simulink model "Model_MPC"  (R2024b)
settings: Solver=FixedStepAuto  StartTime=0.0  StopTime=10  RelTol=1e-3
undefined symbols (not defined in the file): Aa, Ba, Ca, Dm, Eyflat, Fq, Gq, k_3165_plant, k_3166_plant, L, N, qp_iter, Qref, REF_p, REF_q, tau_3165_plant, tau_3166_plant, Ts, umax, Vc_3165, Vc_3166, w, w_eps, X, x0, Y, Z
libraries: sm_lib x13, nesl_utility x5
settings Model: Creator=Giuliano Livi  LastModifiedBy=Giuliano Livi

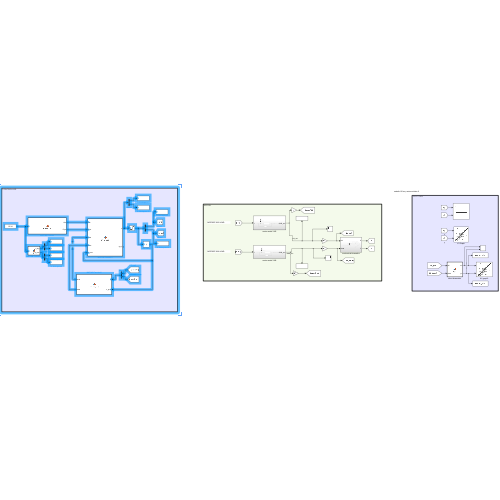
[thumbnail: Simulink's stored preview of the top-level diagram]
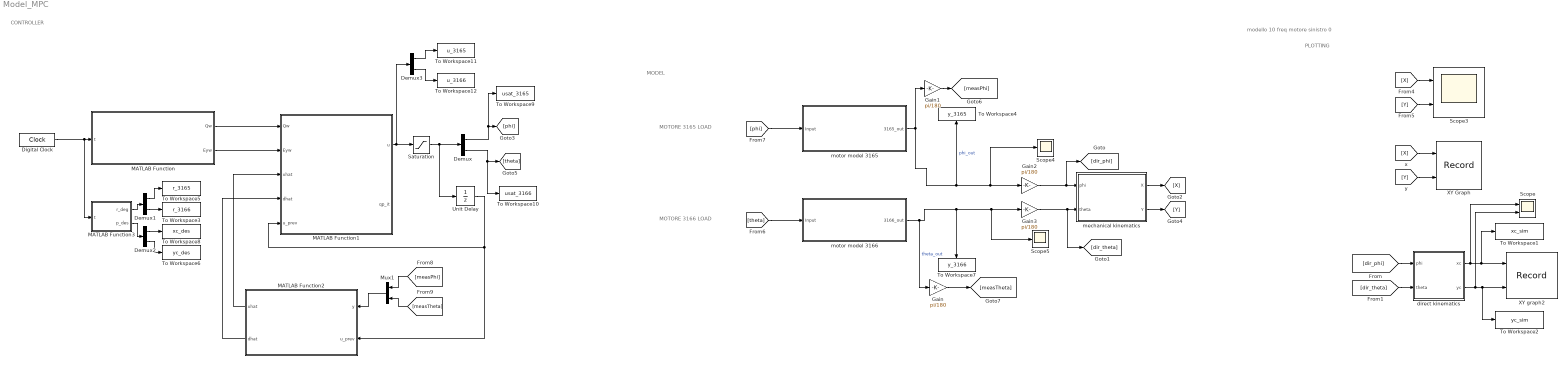
== system Model_MPC ==
  note: CONTROLLER
  note: PLOTTING
  note: MODEL
  note: MOTORE 3165 LOAD
  note: modello 10 freq motore sinistro 0
  note: MOTORE 3166 LOAD
  Demux{,1..3} (4 alike) : Demux  Outputs=2
  Digital Clock : DigitalClock  SampleTime=Ts
  Gain{,1..3} (4 alike) : Gain  Gain=pi/180
  MATLAB Function : MATLAB Function  TreatAsAtomicUnit=on
  MATLAB Function1 : MATLAB Function  TreatAsAtomicUnit=on
  MATLAB Function2 : MATLAB Function  TreatAsAtomicUnit=on
  MATLAB Function3 : MATLAB Function  TreatAsAtomicUnit=on
  Mux1 : Mux  Inputs=2
  Saturation : Saturate  UpperLimit=6  LowerLimit=-6
  Scope : Scope  NumInputPorts=2
  Scope3 : Scope  NumInputPorts=2
  Scope4 : Scope
  Scope5 : Scope
  To Workspace1 : ToWorkspace  VariableName=xc_sim  SaveFormat=Timeseries  SampleTime=0.002
  To Workspace10 : ToWorkspace  VariableName=usat_3166  SaveFormat=Timeseries  SampleTime=0.002
  To Workspace11 : ToWorkspace  VariableName=u_3165  SaveFormat=Timeseries  SampleTime=0.002
  To Workspace12 : ToWorkspace  VariableName=u_3166  SaveFormat=Timeseries  SampleTime=0.002
  To Workspace2 : ToWorkspace  VariableName=yc_sim  SaveFormat=Timeseries  SampleTime=0.002
  To Workspace3 : ToWorkspace  VariableName=r_3166  SaveFormat=Timeseries  SampleTime=0.002
  To Workspace4 : ToWorkspace  VariableName=y_3165  SaveFormat=Timeseries  SampleTime=0.002
  To Workspace5 : ToWorkspace  VariableName=r_3165  SaveFormat=Timeseries  SampleTime=0.002
  To Workspace6 : ToWorkspace  VariableName=yc_des  SaveFormat=Timeseries  SampleTime=0.002
  To Workspace7 : ToWorkspace  VariableName=y_3166  SaveFormat=Timeseries  SampleTime=0.002
  To Workspace8 : ToWorkspace  VariableName=xc_des  SaveFormat=Timeseries  SampleTime=0.002
  To Workspace9 : ToWorkspace  VariableName=usat_3165  SaveFormat=Timeseries  SampleTime=0.002
  Unit Delay : UnitDelay  SampleTime=Ts  HasFrameUpgradeWarning=on
  XY Graph : Record  FileSettingsInternal="{\"entries\":[{\"content\":{\"excelSettings\":{\"content\":{},\"type\":\"Streamout.ExcelSettings\"}},\"type\":\"Streamout.FileSettingStorage\",\"uuid\":\"\"}],\"packageUris\":[\"http:\\/\\/schema.mathworks.com\\/mf0\\/streamout_blocks\\/R2020a\"],\"version\":\"1.0\"}"  Layout=[1 1]  SignalsInternal="{\"entries\":[{\"content\":{\"signals\":[{\"content\":{\"blockPath\":[],\"dimensions\":[1],\"domain\":\"\",\"lineColor\":\"#a2142f\",\"plots\":[ 1 ],\"port\":1,\"sid\":[\"\"],\"signalID\":1,\"signalName\":\"x\"},\"type\":\"RecordBlkView.Signal\",\"uuid\":\"\"},{\"content\":{\"blockPath\":[],\"dimensions\":[1],\"domain\":\"\",\"lineColor\":\"#139fff\",\"plots\":[ 1 ],\"port\":2,\"sid\":[\"\"],\"signalID\":2,\"signalName\":\"y\"},\"type\":\"RecordBlkView.Signal\",\"uuid\":\"\"}]},\"type\":\"RecordBlkView.InputSignals\",\"uuid\":\"\"}],\"packageUris\":[\"http:\\/\\/schema.mathworks.com\\/mf0\\/streamout_blocks\\/R2020a\"],\"version\":\"1.0\"}"  VisualizationBindings="{\"xyplotplugin\":{\"info\":[{\"series\":[{\"bindingParametersList\":[{\"parameter\":\"X-Axis\",\"signalID\":1,\"signalName\":\"x\"},{\"parameter\":\"Y-Axis\",\"signalID\":2,\"signalName\":\"y\"}],\"seriesID\":0}],\"subplotID\":1}]}}"  CompatibilityTag=XY
  XY graph2 : Record  FileSettingsInternal="{\"entries\":[{\"content\":{\"excelSettings\":{\"content\":{},\"type\":\"Streamout.ExcelSettings\"}},\"type\":\"Streamout.FileSettingStorage\",\"uuid\":\"\"}],\"packageUris\":[\"http:\\/\\/schema.mathworks.com\\/mf0\\/streamout_blocks\\/R2020a\"],\"version\":\"1.0\"}"  Layout=[1 1]  SignalsInternal="{\"entries\":[{\"content\":{\"signals\":[{\"content\":{\"blockPath\":[],\"dimensions\":[1],\"domain\":\"\",\"lineColor\":\"#a2142f\",\"lineWidth\":2,\"plots\":[ 1 ],\"port\":1,\"sid\":[\"\"],\"signalID\":1,\"signalName\":\"direct kinematics:1\"},\"type\":\"RecordBlkView.Signal\",\"uuid\":\"\"},{\"content\":{\"blockPath\":[],\"dimensions\":[1],\"domain\":\"\",\"lineColor\":\"#139fff\",\"lineWidth\":2,\"plots\":[ 1 ],\"port\":2,\"sid\":[\"\"],\"signalID\":2,\"signalName\":\"direct kinematics:2\"},\"type\":\"RecordBlkView.Signal\",\"uuid\":\"\"}]},\"type\":\"RecordBlkView.InputSignals\",\"uuid\":\"\"}],\"packageUris\":[\"http:\\/\\/schema.mathworks.com\\/mf0\\/streamout_blocks\\/R2020a\"],\"version\":\"1.0\"}"  VisualizationBindings="{\"xyplotplugin\":{\"info\":[{\"series\":[{\"bindingParametersList\":[{\"parameter\":\"X-Axis\",\"signalID\":1,\"signalName\":\"direct kinematics:1\"},{\"parameter\":\"Y-Axis\",\"signalID\":2,\"signalName\":\"direct kinematics:2\"}],\"seriesID\":0},{\"bindingParametersList\":[{\"parameter\":\"X-Axis\",\"signalID\":1,\"signalName\":\"direct kinematics:1\"},{\"parameter\":\"Y-Axis\",\"signalID\":2,\"signalName\":\"direct kinematics:2\"}],\"seriesID\":1}],\"subplotID\":1}]}}"  CompatibilityTag=XY
  direct kinematics : MATLAB Function  TreatAsAtomicUnit=on  SystemSampleTime=0.002
  mechanical kinematics : Subsystem
  motor model 3165 : Subsystem
  motor model 3166 : Subsystem
  wires:
  Gain2/1 -> mechanical kinematics/1(phi), [dir_phi]
  [X] -> Scope3/1
  [X] -> XY Graph/1
  direct kinematics/2(yc) -> Scope/2, To Workspace2/1, XY graph2/2
  [dir_theta] -> direct kinematics/2(theta)
  motor model 3166/1(3166_out) -> Gain/1, To Workspace7/1, Gain3/1, Scope5/1  "theta_out"
  direct kinematics/1(xc) -> Scope/1, To Workspace1/1, XY graph2/1
  mechanical kinematics/2(Y) -> [Y]
  Gain3/1 -> [dir_theta], mechanical kinematics/2(theta)
  motor model 3165/1(3165_out) -> Gain2/1, Scope4/1, To Workspace4/1, Gain1/1  "phi_out"
  [Y] -> Scope3/2
  mechanical kinematics/1(X) -> [X]
  [phi] -> motor model 3165/1(Input)
  [Y] -> XY Graph/2
  [dir_phi] -> direct kinematics/1(phi)
  [theta] -> motor model 3166/1(Input)
  Digital Clock/1 -> MATLAB Function3/1(t), MATLAB Function/1(t)
  MATLAB Function/2(Eyw) -> MATLAB Function1/2(Eyw)
  MATLAB Function2/1(xhat) -> MATLAB Function1/3(xhat)
  MATLAB Function2/2(dhat) -> MATLAB Function1/4(dhat)
  MATLAB Function1/1(u) -> Saturation/1, Demux3/1
  Saturation/1 -> Unit Delay/1, Demux/1
  Demux/1 -> To Workspace9/1, [phi]
  Demux/2 -> To Workspace10/1, [theta]
  MATLAB Function/1(Qw) -> MATLAB Function1/1(Qw)
  Mux1/1 -> MATLAB Function2/1(y)
  [measPhi] -> Mux1/1
  [measTheta] -> Mux1/2
  Unit Delay/1 -> MATLAB Function2/2(u_prev), MATLAB Function1/5(u_prev)
  Gain/1 -> [measTheta]
  Gain1/1 -> [measPhi]
  MATLAB Function3/1(r_deg) -> Demux1/1
  Demux1/1 -> To Workspace5/1
  Demux1/2 -> To Workspace3/1
  MATLAB Function3/2(p_des) -> Demux2/1
  Demux2/1 -> To Workspace8/1
  Demux2/2 -> To Workspace6/1
  Demux3/1 -> To Workspace11/1
  Demux3/2 -> To Workspace12/1

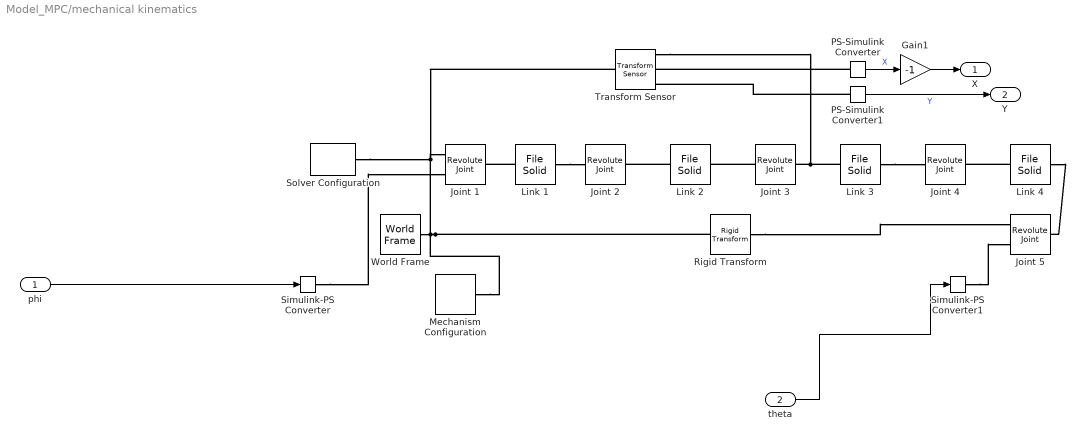
== system Model_MPC/mechanical kinematics ==
  phi : Inport
  theta : Inport  Port=2
  Gain1 : Gain  Gain=-1
  Joint 1 : sm_lib/Joints/Revolute Joint  JointMode=Normal  CompositeWrenchDir=FollowerOnBase  CompositeWrenchFrame=BaseFrame  SenseConstraintForce=off  SenseConstraintTorque=off  SenseTotalForce=off  SenseTotalTorque=off  PositionTargetSpecify=off  PositionTargetPriority=High  PositionTargetValue=0  PositionTargetValueUnits=deg  VelocityTargetSpecify=off  VelocityTargetPriority=High  VelocityTargetValue=0  VelocityTargetValueUnits=deg/s  EquilibriumPosition=0  EquilibriumPositionUnits=deg  SpringStiffness=0  SpringStiffnessUnits=N*m/deg  DampingCoefficient=0  DampingCoefficientUnits=N*m/(deg/s)  LowerLimitSpecify=off  LowerLimitBound=-90  LowerLimitBoundUnits=deg  LowerLimitStiffness=1e4  LowerLimitStiffnessUnits=N*m/deg  LowerLimitDamping=10  LowerLimitDampingUnits=N*m/(deg/s)  LowerLimitTransitionRegionWidth=0.1  LowerLimitTransitionRegionWidthUnits=deg  UpperLimitSpecify=off  UpperLimitBound=90  UpperLimitBoundUnits=deg  UpperLimitStiffness=1e4  UpperLimitStiffnessUnits=N*m/deg  UpperLimitDamping=10  UpperLimitDampingUnits=N*m/(deg/s)  UpperLimitTransitionRegionWidth=0.1  UpperLimitTransitionRegionWidthUnits=deg  TorqueActuationMode=ComputedTorque  MotionActuationMode=InputMotion  SensePosition=off  SenseVelocity=off  SenseAcceleration=off  SenseTorqueForce=off  SenseLowerLimitTorqueForce=off  SenseUpperLimitTorqueForce=off
  Joint 2 : sm_lib/Joints/Revolute Joint  JointMode=Normal  CompositeWrenchDir=FollowerOnBase  CompositeWrenchFrame=BaseFrame  SenseConstraintForce=off  SenseConstraintTorque=off  SenseTotalForce=off  SenseTotalTorque=off  PositionTargetSpecify=off  PositionTargetPriority=High  PositionTargetValue=90  PositionTargetValueUnits=deg  VelocityTargetSpecify=off  VelocityTargetPriority=High  VelocityTargetValue=0  VelocityTargetValueUnits=deg/s  EquilibriumPosition=0  EquilibriumPositionUnits=deg  SpringStiffness=0  SpringStiffnessUnits=N*m/deg  DampingCoefficient=0  DampingCoefficientUnits=N*m/(deg/s)  LowerLimitSpecify=off  LowerLimitBound=-90  LowerLimitBoundUnits=deg  LowerLimitStiffness=1e4  LowerLimitStiffnessUnits=N*m/deg  LowerLimitDamping=10  LowerLimitDampingUnits=N*m/(deg/s)  LowerLimitTransitionRegionWidth=0.1  LowerLimitTransitionRegionWidthUnits=deg  UpperLimitSpecify=off  UpperLimitBound=90  UpperLimitBoundUnits=deg  UpperLimitStiffness=1e4  UpperLimitStiffnessUnits=N*m/deg  UpperLimitDamping=10  UpperLimitDampingUnits=N*m/(deg/s)  UpperLimitTransitionRegionWidth=0.1  UpperLimitTransitionRegionWidthUnits=deg  TorqueActuationMode=NoTorque  MotionActuationMode=ComputedMotion  SensePosition=off  SenseVelocity=off  SenseAcceleration=off  SenseTorqueForce=off  SenseLowerLimitTorqueForce=off  SenseUpperLimitTorqueForce=off
  Joint 3 : sm_lib/Joints/Revolute Joint  JointMode=Normal  CompositeWrenchDir=FollowerOnBase  CompositeWrenchFrame=BaseFrame  SenseConstraintForce=off  SenseConstraintTorque=off  SenseTotalForce=off  SenseTotalTorque=off  PositionTargetSpecify=off  PositionTargetPriority=High  PositionTargetValue=0  PositionTargetValueUnits=deg  VelocityTargetSpecify=off  VelocityTargetPriority=High  VelocityTargetValue=0  VelocityTargetValueUnits=deg/s  EquilibriumPosition=0  EquilibriumPositionUnits=deg  SpringStiffness=0  SpringStiffnessUnits=N*m/deg  DampingCoefficient=0  DampingCoefficientUnits=N*m/(deg/s)  LowerLimitSpecify=off  LowerLimitBound=-90  LowerLimitBoundUnits=deg  LowerLimitStiffness=1e4  LowerLimitStiffnessUnits=N*m/deg  LowerLimitDamping=10  LowerLimitDampingUnits=N*m/(deg/s)  LowerLimitTransitionRegionWidth=0.1  LowerLimitTransitionRegionWidthUnits=deg  UpperLimitSpecify=off  UpperLimitBound=90  UpperLimitBoundUnits=deg  UpperLimitStiffness=1e4  UpperLimitStiffnessUnits=N*m/deg  UpperLimitDamping=10  UpperLimitDampingUnits=N*m/(deg/s)  UpperLimitTransitionRegionWidth=0.1  UpperLimitTransitionRegionWidthUnits=deg  TorqueActuationMode=NoTorque  MotionActuationMode=ComputedMotion  SensePosition=off  SenseVelocity=off  SenseAcceleration=off  SenseTorqueForce=off  SenseLowerLimitTorqueForce=off  SenseUpperLimitTorqueForce=off
  Joint 4 : sm_lib/Joints/Revolute Joint  JointMode=Normal  CompositeWrenchDir=FollowerOnBase  CompositeWrenchFrame=BaseFrame  SenseConstraintForce=off  SenseConstraintTorque=off  SenseTotalForce=off  SenseTotalTorque=off  PositionTargetSpecify=off  PositionTargetPriority=High  PositionTargetValue=0  PositionTargetValueUnits=deg  VelocityTargetSpecify=off  VelocityTargetPriority=High  VelocityTargetValue=0  VelocityTargetValueUnits=deg/s  EquilibriumPosition=0  EquilibriumPositionUnits=deg  SpringStiffness=0  SpringStiffnessUnits=N*m/deg  DampingCoefficient=0  DampingCoefficientUnits=N*m/(deg/s)  LowerLimitSpecify=off  LowerLimitBound=-90  LowerLimitBoundUnits=deg  LowerLimitStiffness=1e4  LowerLimitStiffnessUnits=N*m/deg  LowerLimitDamping=10  LowerLimitDampingUnits=N*m/(deg/s)  LowerLimitTransitionRegionWidth=0.1  LowerLimitTransitionRegionWidthUnits=deg  UpperLimitSpecify=off  UpperLimitBound=90  UpperLimitBoundUnits=deg  UpperLimitStiffness=1e4  UpperLimitStiffnessUnits=N*m/deg  UpperLimitDamping=10  UpperLimitDampingUnits=N*m/(deg/s)  UpperLimitTransitionRegionWidth=0.1  UpperLimitTransitionRegionWidthUnits=deg  TorqueActuationMode=NoTorque  MotionActuationMode=ComputedMotion  SensePosition=off  SenseVelocity=off  SenseAcceleration=off  SenseTorqueForce=off  SenseLowerLimitTorqueForce=off  SenseUpperLimitTorqueForce=off
  Joint 5 : sm_lib/Joints/Revolute Joint  JointMode=Normal  CompositeWrenchDir=FollowerOnBase  CompositeWrenchFrame=BaseFrame  SenseConstraintForce=off  SenseConstraintTorque=off  SenseTotalForce=off  SenseTotalTorque=off  PositionTargetSpecify=off  PositionTargetPriority=High  PositionTargetValue=0  PositionTargetValueUnits=deg  VelocityTargetSpecify=off  VelocityTargetPriority=High  VelocityTargetValue=0  VelocityTargetValueUnits=deg/s  EquilibriumPosition=0  EquilibriumPositionUnits=deg  SpringStiffness=0  SpringStiffnessUnits=N*m/deg  DampingCoefficient=0  DampingCoefficientUnits=N*m/(deg/s)  LowerLimitSpecify=off  LowerLimitBound=-90  LowerLimitBoundUnits=deg  LowerLimitStiffness=1e4  LowerLimitStiffnessUnits=N*m/deg  LowerLimitDamping=10  LowerLimitDampingUnits=N*m/(deg/s)  LowerLimitTransitionRegionWidth=0.1  LowerLimitTransitionRegionWidthUnits=deg  UpperLimitSpecify=off  UpperLimitBound=90  UpperLimitBoundUnits=deg  UpperLimitStiffness=1e4  UpperLimitStiffnessUnits=N*m/deg  UpperLimitDamping=10  UpperLimitDampingUnits=N*m/(deg/s)  UpperLimitTransitionRegionWidth=0.1  UpperLimitTransitionRegionWidthUnits=deg  TorqueActuationMode=ComputedTorque  MotionActuationMode=InputMotion  SensePosition=off  SenseVelocity=off  SenseAcceleration=off  SenseTorqueForce=off  SenseLowerLimitTorqueForce=off  SenseUpperLimitTorqueForce=off
  Link 1 : sm_lib/Body Elements/File Solid  ExtGeomFileName=link.step  UnitType=FromFile  ExtGeomFileUnits=m  StepReaderType=HEX  ExportConvexHullGeometry=off  InertiaType=CalculateFromGeometry  BasedOnType=Mass  Density=1000  DensityUnits=kg/m^3  Mass=0.065  MassUnits=kg  CenterOfMass=[0 0 0]  CenterOfMassUnits=m  MomentsOfInertia=[1 1 1]  MomentsOfInertiaUnits=kg*m^2  ProductsOfInertia=[0 0 0]  ProductsOfInertiaUnits=kg*m^2  GraphicType=FromGeometry  MarkerShape=Sphere  MarkerSize=10  GraphicVisPropType=SimpleVisualProperties  GraphicDiffuseColor=[0.5 0.5 0.5]  GraphicOpacity=1  GraphicSpecularColor=[0.5 0.5 0.5 1.0]  GraphicAmbientColor=[0.15 0.15 0.15 1.0]  GraphicEmissiveColor=[0.0 0.0 0.0 1.0]  GraphicShininess=75  DoExposeReferenceFrame=off  SerializedFrames=<Frames><Frame><Id>Frame1</Id><Value><Name>F1</Name><Origin><Source>GeometricFeature</Source><FeatureName>cylindrical surface 1</FeatureName></Origin><PrimaryAxis><DefinedDirection>+Z</DefinedDirection><Source>ReferenceFrame</Source><SourceDirection>+Z</SourceDirection><FeatureName></FeatureName></PrimaryAxis><SecondaryAxis><DefinedDirection>+Y</DefinedDirection><Source>ReferenceFrame</Source><SourceDirection>+X</SourceDirection><FeatureName></FeatureName></SecondaryAxis></Value></Frame><Frame><Id>Frame2</Id><Value><Name>F2</Name><Origin><Source>GeometricFeature</Source><FeatureName>cylindrical surface 2</FeatureName></Origin><PrimaryAxis><DefinedDirection>+Z</DefinedDirection><Source>ReferenceFrame</Source><SourceDirection>+Z</SourceDirection><FeatureName></FeatureName></PrimaryAxis><SecondaryAxis><DefinedDirection>+X</DefinedDirection><Source>ReferenceFrame</Source><SourceDirection>+X</SourceDirection><FeatureName></FeatureName></SecondaryAxis></Value></Frame></Frames>
  Link 2 : sm_lib/Body Elements/File Solid  ExtGeomFileName=link.step  UnitType=FromFile  ExtGeomFileUnits=m  StepReaderType=HEX  ExportConvexHullGeometry=off  InertiaType=CalculateFromGeometry  BasedOnType=Mass  Density=1000  DensityUnits=kg/m^3  Mass=0.065  MassUnits=kg  CenterOfMass=[0 0 0]  CenterOfMassUnits=m  MomentsOfInertia=[1 1 1]  MomentsOfInertiaUnits=kg*m^2  ProductsOfInertia=[0 0 0]  ProductsOfInertiaUnits=kg*m^2  GraphicType=FromGeometry  MarkerShape=Sphere  MarkerSize=10  GraphicVisPropType=SimpleVisualProperties  GraphicDiffuseColor=[0.5 0.5 0.5]  GraphicOpacity=1  GraphicSpecularColor=[0.5 0.5 0.5 1.0]  GraphicAmbientColor=[0.15 0.15 0.15 1.0]  GraphicEmissiveColor=[0.0 0.0 0.0 1.0]  GraphicShininess=75  DoExposeReferenceFrame=off  SerializedFrames=<Frames><Frame><Id>Frame1</Id><Value><Name>F1</Name><Origin><Source>GeometricFeature</Source><FeatureName>cylindrical surface 1</FeatureName></Origin><PrimaryAxis><DefinedDirection>+Z</DefinedDirection><Source>ReferenceFrame</Source><SourceDirection>+Z</SourceDirection><FeatureName></FeatureName></PrimaryAxis><SecondaryAxis><DefinedDirection>+X</DefinedDirection><Source>ReferenceFrame</Source><SourceDirection>+X</SourceDirection><FeatureName></FeatureName></SecondaryAxis></Value></Frame><Frame><Id>Frame2</Id><Value><Name>F2</Name><Origin><Source>GeometricFeature</Source><FeatureName>cylindrical surface 2</FeatureName></Origin><PrimaryAxis><DefinedDirection>+Z</DefinedDirection><Source>ReferenceFrame</Source><SourceDirection>+Z</SourceDirection><FeatureName></FeatureName></PrimaryAxis><SecondaryAxis><DefinedDirection>+X</DefinedDirection><Source>ReferenceFrame</Source><SourceDirection>+X</SourceDirection><FeatureName></FeatureName></SecondaryAxis></Value></Frame></Frames>
  Link 3 : sm_lib/Body Elements/File Solid  ExtGeomFileName=link.step  UnitType=FromFile  ExtGeomFileUnits=m  StepReaderType=HEX  ExportConvexHullGeometry=off  InertiaType=CalculateFromGeometry  BasedOnType=Mass  Density=1000  DensityUnits=kg/m^3  Mass=0.065  MassUnits=kg  CenterOfMass=[0 0 0]  CenterOfMassUnits=m  MomentsOfInertia=[1 1 1]  MomentsOfInertiaUnits=kg*m^2  ProductsOfInertia=[0 0 0]  ProductsOfInertiaUnits=kg*m^2  GraphicType=FromGeometry  MarkerShape=Sphere  MarkerSize=10  GraphicVisPropType=SimpleVisualProperties  GraphicDiffuseColor=[0.5 0.5 0.5]  GraphicOpacity=1  GraphicSpecularColor=[0.5 0.5 0.5 1.0]  GraphicAmbientColor=[0.15 0.15 0.15 1.0]  GraphicEmissiveColor=[0.0 0.0 0.0 1.0]  GraphicShininess=75  DoExposeReferenceFrame=off  SerializedFrames=<Frames><Frame><Id>Frame1</Id><Value><Name>F1</Name><Origin><Source>GeometricFeature</Source><FeatureName>cylindrical surface 1</FeatureName></Origin><PrimaryAxis><DefinedDirection>+Z</DefinedDirection><Source>ReferenceFrame</Source><SourceDirection>+Z</SourceDirection><FeatureName></FeatureName></PrimaryAxis><SecondaryAxis><DefinedDirection>+X</DefinedDirection><Source>ReferenceFrame</Source><SourceDirection>+X</SourceDirection><FeatureName></FeatureName></SecondaryAxis></Value></Frame><Frame><Id>Frame2</Id><Value><Name>F2</Name><Origin><Source>GeometricFeature</Source><FeatureName>cylindrical surface 2</FeatureName></Origin><PrimaryAxis><DefinedDirection>+Z</DefinedDirection><Source>ReferenceFrame</Source><SourceDirection>+Z</SourceDirection><FeatureName></FeatureName></PrimaryAxis><SecondaryAxis><DefinedDirection>+X</DefinedDirection><Source>ReferenceFrame</Source><SourceDirection>+X</SourceDirection><FeatureName></FeatureName></SecondaryAxis></Value></Frame></Frames>
  Link 4 : sm_lib/Body Elements/File Solid  ExtGeomFileName=link.step  UnitType=FromFile  ExtGeomFileUnits=m  StepReaderType=HEX  ExportConvexHullGeometry=off  InertiaType=CalculateFromGeometry  BasedOnType=Mass  Density=1000  DensityUnits=kg/m^3  Mass=0.065  MassUnits=kg  CenterOfMass=[0 0 0]  CenterOfMassUnits=m  MomentsOfInertia=[1 1 1]  MomentsOfInertiaUnits=kg*m^2  ProductsOfInertia=[0 0 0]  ProductsOfInertiaUnits=kg*m^2  GraphicType=FromGeometry  MarkerShape=Sphere  MarkerSize=10  GraphicVisPropType=SimpleVisualProperties  GraphicDiffuseColor=[0.5 0.5 0.5]  GraphicOpacity=1  GraphicSpecularColor=[0.5 0.5 0.5 1.0]  GraphicAmbientColor=[0.15 0.15 0.15 1.0]  GraphicEmissiveColor=[0.0 0.0 0.0 1.0]  GraphicShininess=75  DoExposeReferenceFrame=off  SerializedFrames=<Frames><Frame><Id>Frame1</Id><Value><Name>F1</Name><Origin><Source>GeometricFeature</Source><FeatureName>cylindrical surface 1</FeatureName></Origin><PrimaryAxis><DefinedDirection>+Z</DefinedDirection><Source>ReferenceFrame</Source><SourceDirection>+Z</SourceDirection><FeatureName></FeatureName></PrimaryAxis><SecondaryAxis><DefinedDirection>+X</DefinedDirection><Source>ReferenceFrame</Source><SourceDirection>+X</SourceDirection><FeatureName></FeatureName></SecondaryAxis></Value></Frame><Frame><Id>Frame2</Id><Value><Name>F2</Name><Origin><Source>GeometricFeature</Source><FeatureName>cylindrical surface 2</FeatureName></Origin><PrimaryAxis><DefinedDirection>+Z</DefinedDirection><Source>ReferenceFrame</Source><SourceDirection>+Z</SourceDirection><FeatureName></FeatureName></PrimaryAxis><SecondaryAxis><DefinedDirection>+X</DefinedDirection><Source>ReferenceFrame</Source><SourceDirection>+X</SourceDirection><FeatureName></FeatureName></SecondaryAxis></Value></Frame></Frames>
  Mechanism Configuration : sm_lib/Utilities/Mechanism Configuration  UniformGravity=Constant  GravityVector=[0 0 -9.80665]  GravityVectorUnits=m/s^2  LinearizationDelta=0.001  JointModeTransitionNonlinearIterations=2
  PS-Simulink Converter : nesl_utility/PS-Simulink Converter  PhysicalDomain=network_engine_domain  SubClassName=ps_output  LeftPortType=input  RightPortType=output  PseudoPeriodic=off  Frequencies=[]  VectorFormat=inherit  Unit=inherit  AffineConversion=off
  PS-Simulink Converter1 : nesl_utility/PS-Simulink Converter  PhysicalDomain=network_engine_domain  SubClassName=ps_output  LeftPortType=input  RightPortType=output  PseudoPeriodic=off  Frequencies=[]  VectorFormat=inherit  Unit=inherit  AffineConversion=off
  Rigid Transform : sm_lib/Frames and Transforms/Rigid Transform  RotationMethod=None  FollAlignAxisA=+X  BaseAlignAxisA=+Y  FollAlignAxisB=+Y  BaseAlignAxisB=+Z  RotationStandardAxis=+Z  RotationAngle=0  RotationAngleUnits=deg  RotationArbitraryAxis=[0 0 1]  RotationSequenceAxes=FollowerAxes  RotationSequence=XYX  RotationSequenceAngles=[0 0 0]  RotationSequenceAnglesUnits=deg  RotationMatrix=[1 0 0;0 1 0;0 0 1]  Quaternion=[1 0 0 0]  TranslationMethod=Cartesian  TranslationCartesianOffset=[0 0.254 0]  TranslationCartesianOffsetUnits=m  TranslationStandardAxis=+Z  TranslationStandardOffset=0  TranslationStandardOffsetUnits=m  TranslationROffset=0  TranslationROffsetUnits=m  TranslationThetaOffset=0  TranslationThetaOffsetUnits=deg  TranslationZOffset=0  TranslationZOffsetUnits=m
  Simulink-PS Converter : nesl_utility/Simulink-PS Converter  PhysicalDomain=network_engine_domain  SubClassName=ps_input  LeftPortType=input  RightPortType=output  PseudoPeriodic=off  Frequencies=[]  NoiseDistribution=none  NoiseParameters=[]  Unit=rad  AffineConversion=off  FilteringAndDerivatives=filter  SimscapeFilterOrder=2  InputFilterTimeConstant=0.001  UdotUserProvided=0
  Simulink-PS Converter1 : nesl_utility/Simulink-PS Converter  PhysicalDomain=network_engine_domain  SubClassName=ps_input  LeftPortType=input  RightPortType=output  PseudoPeriodic=off  Frequencies=[]  NoiseDistribution=none  NoiseParameters=[]  Unit=rad  AffineConversion=off  FilteringAndDerivatives=filter  SimscapeFilterOrder=2  InputFilterTimeConstant=0.001  UdotUserProvided=0
  Solver Configuration : nesl_utility/Solver Configuration  PhysicalDomain=network_engine_domain  SubClassName=solver  LeftPortType=input  RightPortType=generic  Tones=[]  Harmonics=[]  SimulateNoise=off  Profile=off  UseLocalSampling=off  EnableSwitchedLinearOptims=on  FrequencyDomain=off  UseCCode=off  RelTol=0.001  AbsTol=0.001  MinStep=1e-09  ToWorkspace=off  RevertToSquareIcSolve=off  NumHomotopyIterations=100  PhasorMode=off  PhasorModeNumHarmonics=1  ConsistencySolver=NEWTON_XTOL_AFTER_FTOL  IndexReductionMethod=DerivativeReplacement  DoDC=on  ResidualTolerance=1e-09  ConsistencyTolSource=GLOBAL  ConsistencyAbsTol=0.001  ConsistencyRelTol=0.001  ConsistencyTolFactor=0.001  UseLocalSolver=off  LocalSolverChoice=NE_BACKWARD_EULER_ADVANCER  ResolveIndetEquations=on  FunctionEvalNumThread=1  LocalSolverSampleTime=0.002  DoFixedCost=off  MaxNonlinIter=3  MaxModeIter=2  ComputeImpulses=off  ImpulseIterations=2  LinearAlgebra=auto  LinearAlgebraNumThread=0  EquationFormulation=NE_TIME_EF  DelaysMemoryBudget=1024  AutomaticFiltering=on  FilteringTimeConstant=0.001  PartitionStorageMethod=AS_NEEDED  PartitionMemoryBudget=1024  PartitionMethod=ROBUST  MultibodyUseLocalSolver=off  MultibodyLocalSolverChoice=ODE2  MultibodyLocalSolverSampleTime=0.002
  Transform Sensor : sm_lib/Frames and Transforms/Transform Sensor  MeasurementFrame=World  RotationSequence=XYX  SenseAngle=off  SenseAxis=off  SenseQ=off  SenseR=off  SenseRotationSequence=off  SenseOmegaX=off  SenseOmegaY=off  SenseOmegaZ=off  SenseOmega=off  SenseQDot=off  SenseRDot=off  SenseRotationSequenceDot=off  SenseAlphaX=off  SenseAlphaY=off  SenseAlphaZ=off  SenseAlpha=off  SenseQDDot=off  SenseRDDot=off  SenseX=on  SenseY=on  SenseZ=off  SenseXYZ=off  SenseRad=off  SenseAzim=off  SenseDist=off  SenseInc=off  SenseXDot=off  SenseYDot=off  SenseZDot=off  SenseXYZDot=off  SenseRadDot=off  SenseAzimDot=off  SenseDistDot=off  SenseIncDot=off  SenseXDDot=off  SenseYDDot=off  SenseZDDot=off  SenseXYZDDot=off  SenseRadDDot=off  SenseAzimDDot=off  SenseDistDDot=off  SenseIncDDot=off
  World Frame : sm_lib/Frames and Transforms/World Frame
  X : Outport
  Y : Outport  Port=2
  wires:
  theta/1 -> Simulink-PS Converter1/1
  phi/1 -> Simulink-PS Converter/1
  PS-Simulink Converter1/1 -> Y/1  "Y"
  PS-Simulink Converter/1 -> Gain1/1  "X"
  Gain1/1 -> X/1
  connections:
  World Frame/RConn1 -- Rigid Transform/LConn1 -- Transform Sensor/LConn1 -- Joint 1/LConn1 -- Solver Configuration/RConn1 -- Mechanism Configuration/RConn1
  Joint 3/LConn1 -- Link 2/RConn1
  Link 3/LConn1 -- Transform Sensor/RConn1 -- Joint 3/RConn1
  Simulink-PS Converter1/RConn1 -- Joint 5/LConn2
  Rigid Transform/RConn1 -- Joint 5/LConn1
  Link 3/RConn1 -- Joint 4/LConn1
  Link 1/RConn1 -- Joint 2/LConn1
  Link 4/LConn1 -- Joint 4/RConn1
  Link 4/RConn1 -- Joint 5/RConn1
  Link 2/LConn1 -- Joint 2/RConn1
  Link 1/LConn1 -- Joint 1/RConn1
  Simulink-PS Converter/RConn1 -- Joint 1/LConn2
  PS-Simulink Converter/LConn1 -- Transform Sensor/RConn2
  PS-Simulink Converter1/LConn1 -- Transform Sensor/RConn3

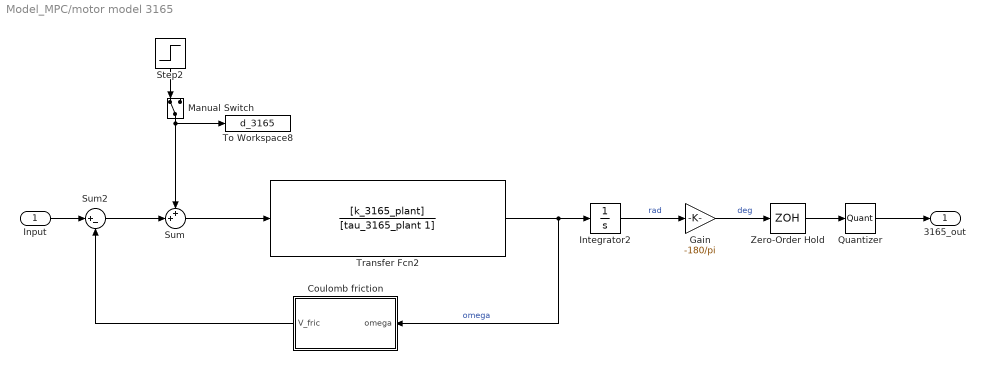
== system Model_MPC/motor model 3165 ==
  Input : Inport
  Coulomb friction : MATLAB Function  TreatAsAtomicUnit=on
  Gain : Gain  Gain=-180/pi
  Integrator2 : Integrator
  Manual Switch : ManualSwitch
  Quantizer : Quantizer  QuantizationInterval=360/4096
  Step2 : Step  Time=5  After=0.5  SampleTime=0
  Sum : Sum  Inputs=++|
  Sum2 : Sum  Inputs=|+-
  To Workspace8 : ToWorkspace  VariableName=d_3165  SaveFormat=Timeseries  SampleTime=-1
  Transfer Fcn2 : TransferFcn  Numerator=[k_3165_plant]  Denominator=[tau_3165_plant 1]
  Zero-Order Hold : ZeroOrderHold  SampleTime=0.002
  3165_out : Outport
  wires:
  Transfer Fcn2/1 -> Coulomb friction/1(omega), Integrator2/1  "omega"
  Integrator2/1 -> Gain/1  "rad"
  Gain/1 -> Zero-Order Hold/1  "deg"
  Quantizer/1 -> 3165_out/1
  Zero-Order Hold/1 -> Quantizer/1
  Manual Switch/1 -> Sum/1, To Workspace8/1
  Input/1 -> Sum2/1
  Sum/1 -> Transfer Fcn2/1
  Sum2/1 -> Sum/2
  Step2/1 -> Manual Switch/1
  Coulomb friction/1(V_fric) -> Sum2/2

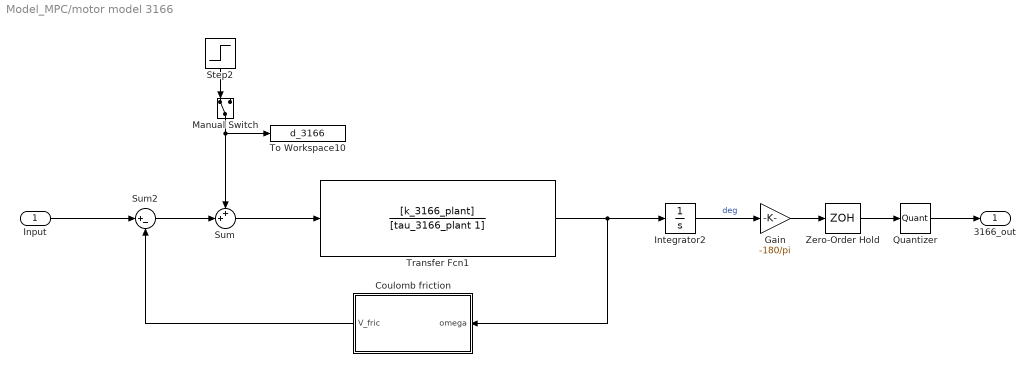
== system Model_MPC/motor model 3166 ==
  Input : Inport
  Coulomb friction : MATLAB Function  TreatAsAtomicUnit=on
  Gain : Gain  Gain=-180/pi
  Integrator2 : Integrator
  Manual Switch : ManualSwitch
  Quantizer : Quantizer  QuantizationInterval=360/4096
  Step2 : Step  Time=5  After=0.5  SampleTime=0
  Sum : Sum  Inputs=++|
  Sum2 : Sum  Inputs=|+-
  To Workspace10 : ToWorkspace  VariableName=d_3166  SaveFormat=Timeseries  SampleTime=-1
  Transfer Fcn1 : TransferFcn  Numerator=[k_3166_plant]  Denominator=[tau_3166_plant 1]
  Zero-Order Hold : ZeroOrderHold  SampleTime=0.002
  3166_out : Outport
  wires:
  Transfer Fcn1/1 -> Coulomb friction/1(omega), Integrator2/1
  Integrator2/1 -> Gain/1  "deg"
  Gain/1 -> Zero-Order Hold/1
  Quantizer/1 -> 3166_out/1
  Zero-Order Hold/1 -> Quantizer/1
  Sum2/1 -> Sum/2
  Step2/1 -> Manual Switch/1
  Input/1 -> Sum2/1
  Coulomb friction/1(V_fric) -> Sum2/2
  Manual Switch/1 -> To Workspace10/1, Sum/1
  Sum/1 -> Transfer Fcn1/1

== matlab function Model_MPC/MATLAB Function1 ==
  data: Qw input; Eyw input; xhat input; u output; dhat input; u_prev input; qp_it output; Fq parameter; Gq parameter; umax parameter; Dm parameter; E0 parameter; qp_iter parameter; w parameter
function [u, qp_it] = mpc_step(Qw, Eyw, xhat, dhat, u_prev, Fq, Gq, umax, Dm, E0, qp_iter, w)
%#codegen
% MATLAB Function block: LTV MPC on contour / lag error, one QP per sample.
% Inputs (signals):
%   xhat   [4x1]  state estimate [phi; dphi; theta; dtheta]        (kalman_step)
%   dhat   [2x1]  input-disturbance estimate [V]                   (kalman_step)
%   Qw     [2xN]  window of q_ref,{k+j} [rad]                         (refWindow)
%   Eyw    [4xN]  window of Ey_{k+j} = [n'; t'] * J  (column-major)  (refWindow)
%   u_prev [2x1]  input applied at the previous sample [V]  (after saturation, Unit Delay)
% Parameters: Fq = mpc.Fq, Gq = mpc.Gq, Dm = mpc.Dm, E0 = mpc.E0, w = mpc.w (struct),
%             umax = mpc.umax, qp_iter = mpc.qp_iter
% Outputs: u [2x1] voltage to apply [V],  qp_it = active-set iterations used
%
% Decision variable V = U + d (the plant sees u + d):  q_pred = Fq*x + Gq*V
%   cost = sum_j [ qc*e_c,j^2 + ql*e_l,j^2 ] + r*|dU|^2
%   e_j = Ey_j * (q_j - q_ref,j),    dU = Dm*V - E0*(u_prev + d)
%   -umax <= u = V - d <= umax   ->   d - umax <= V <= d + umax
 
% Everything is prepared for the solver:

N  = size(Eyw, 2);
nV = size(Gq, 2);
x  = xhat(:);  
d = dhat(:);
 
% 1. Linearized contour/lag error along the horizon:  e = M*V + c
M = zeros(2*N, nV);
c = zeros(2*N, 1);
for j = 1:N
    r2 = 2*j-1:2*j;
    Ej = reshape(Eyw(:,j), 2, 2);
    M(r2, :) = Ej*Gq(r2, :);
    c(r2) = Ej*(Fq(r2,:)*x - Qw(:,j));          % e = Ey*(q_pred - q_ref)
end
Wv = repmat([w.qc; w.ql], N, 1);
 
% 2. QP:  min 0.5*V'*H*V + f'*V   s.t.  lb <= V <= ub
H = 2*(M'*(Wv.*M) + w.r*(Dm'*Dm));
f = 2*(M'*(Wv.*c) - w.r*(Dm'*(E0*(u_prev(:) + d))));
H = 0.5*(H + H');                                  % exact symmetry
lb = repmat(d - umax, nV/2, 1);
ub = repmat(d + umax, nV/2, 1);
 
[V, qp_it] = box_qp(H, f, lb, ub, qp_iter);
 
% 3. Receding horizon: apply only the first move
u = V(1:2) - d;
end
 
%% ------------------------------------------------------------------------
function [U, it] = box_qp(H, f, lb, ub, maxit)
% Exact solver for a small QP with box constraints (primal-dual active set).
% Starts from the unconstrained optimum: if it is feasible (no saturation),
% the answer is exact after one linear solve.
n  = numel(f);
U  = -(H\f);
it = 0;
lo = U < lb;
up = U > ub;
while (any(lo) || any(up)) && it < maxit
    it = it + 1;
    % Solve with the active variables fixed at their bound
    Hm = H;  rhs = -f;
    for i = 1:n
        if lo(i) || up(i)
            Hm(i, :) = 0;  Hm(i, i) = 1;
            if lo(i), rhs(i) = lb(i); else, rhs(i) = ub(i); end
        end
    end
    U = Hm\rhs;
    g = H*U + f;                                   % gradient = minus the multipliers
    % Keep a bound only if the gradient pushes outwards, add the violated ones
    lo_new = (U < lb - 1e-12) | (lo & g > 0);
    up_new = (U > ub + 1e-12) | (up & g < 0);
    if isequal(lo_new, lo) && isequal(up_new, up)
        break;                                     % KKT conditions satisfied
    end
    lo = lo_new;  up = up_new;
end
U = min(max(U, lb), ub);                           % safety clip
end

== matlab function Model_MPC/MATLAB Function ==
  data: t input; Qw output; Eyw output; Qref parameter; Eyflat parameter; N parameter; Ts parameter
function [Qw, Eyw] = refWindow(t, Qref, Eyflat, N, Ts)
%#codegen
% MATLAB Function block: preview window r_{k+1} ... r_{k+N} for the MPC.
%   k      : current sample index, 0-based (input port, e.g. from a counter)
%   Qref   = REF_q   [2 x n]  joint reference [rad]
%   Eyflat = REF_Ey  [4 x n]  contour/lag maps Ey = [n'; t']*J, column-major
%   N      = mpc horizon
%   (Qref, Eyflat, N: declare them as PARAMETERS in the Ports and Data Manager)
% Outputs, one column per horizon step j = 1..N:
%   Qw [2xN] joint reference,  Eyw [4xN] (reshape column j to 2x2 to get Ey_{k+j})
k   = round(t/Ts);                 % sample index (0-based) from the time
nS  = size(Qref, 2);
idx = min(k + (2:N+1), nS);
Qw  = Qref(:, idx);
Eyw = Eyflat(:, idx);
end

== matlab function Model_MPC/motor model 3165/Coulomb friction ==
  data: omega input; V_fric output; Vc_3165 parameter; w_eps parameter
function V_fric = coulomb_friction(omega, Vc_3165, w_eps)
%#codegen
% Coulomb friction as an equivalent voltage at the motor input.
% omega : motor velocity [rad/s] (output of the Transfer Fcn)
% Vc    : Coulomb voltage [V]
% w_eps : width of the smooth transition around zero speed [rad/s]
V_fric = Vc_3165 * tanh(omega / w_eps);
end

== matlab function Model_MPC/direct kinematics ==
  data: phi input; xc output; theta input; yc output
function [xc, yc] = fcn(phi, theta)
l = 0.127;
a = 2 - sin(theta) - cos(phi);
b = cos(theta) - sin(phi);
s = sqrt(a^2 + b^2);
h = l*sqrt(1 - s^2/4);

% Nonlinear forward kinematics of point C
xc = l/2*(2 - sin(theta) + cos(phi)) - h*b/s;
yc = l/2*(cos(theta) + sin(phi))     + h*a/s;

== matlab function Model_MPC/motor model 3166/Coulomb friction ==
  data: omega input; V_fric output; Vc_3166 parameter; w_eps parameter
function V_fric = coulomb_friction(omega, Vc_3166, w_eps)
%#codegen
% Coulomb friction as an equivalent voltage at the motor input.
% omega : motor velocity [rad/s] (output of the Transfer Fcn)
% Vc    : Coulomb voltage [V]
% w_eps : width of the smooth transition around zero speed [rad/s]
V_fric = Vc_3166 * tanh(omega / w_eps);
end

== matlab function Model_MPC/MATLAB Function2 ==
  data: y input; xhat output; u_prev input; dhat output; Aa parameter; Ba parameter; Ca parameter; x0 parameter; L parameter
function [xhat, dhat] = kalman_step(y, u_prev, Aa, Ba, Ca, x0, L)
%#codegen
% MATLAB Function block: steady-state Kalman filter with input-disturbance states.
%   y      [2x1] measured joint angles [rad]  (encoder deg * pi/180)
%   u_prev [2x1] input APPLIED at the previous sample [V] (after the saturation, Unit Delay)
%   Aa, Ba, Ca, L, x0 : PARAMETERS  (est.Aa, est.Ba, est.Ca, est.L, initial state [6x1])
% Outputs (estimate at time k, after using y_k):
%   xhat [4x1] = [phi; dphi; theta; dtheta]     dhat [2x1] input disturbance [V]
% Model: xa = [x; d], x_{k+1} = A x + B (u + d), d_{k+1} = d, y = [phi; theta]
 
persistent xa
if isempty(xa)
    xa = x0;                       % start: robot at home, at rest, no disturbance
else
    xa = Aa*xa + Ba*u_prev;        % time update with the input actually applied at k-1
end
xa = xa + L*(y - Ca*xa);           % measurement update with y_k
 
xhat = xa(1:4);
dhat = xa(5:6);
end

== matlab function Model_MPC/MATLAB Function3 ==
  data: t input; r_deg output; p_des output; REF_q parameter; REF_p parameter; Ts parameter
function [r_deg, p_des] = fcn(t, REF_q, REF_p, Ts)
i = min(round(t/Ts) + 1, size(REF_q, 2));   % current sample (MATLAB index)
r_deg = REF_q(:, i) * 180/pi;               % encoder degrees
p_des = REF_p(:, i);                        % [x; y] desired [m]
end
